simulink model "green_velocity"  (R2021a)
settings: Solver=VariableStepAuto  StartTime=0.0  StopTime=simTime  RelTol=1e-3
InitFcn:
  | gree_wave_velocity_init
values from neighbouring files (symbols this model uses):
  Kd = 0    [gree_wave_velocity_init.m]
  Ki = 51.1361    [gree_wave_velocity_init.m]
  Kp = 490.9572    [gree_wave_velocity_init.m]
  simTime = 1800    [gree_wave_velocity_init.m]
  v2x_traffic_signal = [light;time_fullwave(1:length(t)-1)]'    [gree_wave_velocity_init.m]
libraries: pid_lib x1
settings Model: Creator=srini  LastModifiedBy=srini

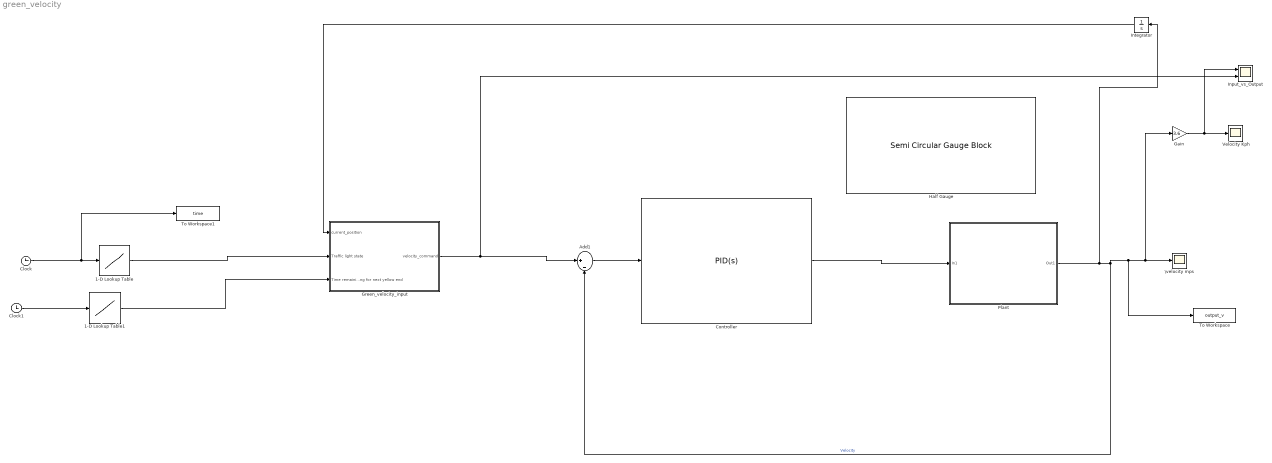
== system green_velocity ==
  1-D Lookup Table : Lookup_n-D  NumberOfTableDimensions=1  BreakpointsForDimension1=t(1:(simTime-1))  Table=v2x_traffic_signal(:,1)  InterpMethod=Nearest  InternalRulePriority=Speed  RndMeth=Simplest  InputSameDT=on
  1-D Lookup Table1 : Lookup_n-D  NumberOfTableDimensions=1  BreakpointsForDimension1=t(1:(simTime-1))  Table=v2x_traffic_signal(:,2)  InternalRulePriority=Speed  RndMeth=Simplest  InputSameDT=on
  Add1 : Sum  Inputs=|+-
  Clock : Clock
  Clock1 : Clock
  Controller : pid_lib/PID Controller  Controller=PID  Form=Parallel  TimeDomain=Continuous-time  UseExternalTs=off  SampleTime=-1  IntegratorMethod=Forward Euler  FilterMethod=Forward Euler  ControllerParametersSource=internal  P=Kp  I=Ki  D=Kd  UseFilter=on  N=100  TunerSelectOption=Transfer Function Based (PID Tuner App)  InitialConditionSource=internal  InitialConditionForIntegrator=0  InitialConditionForFilter=0  DifferentiatorICPrevScaledInput=0  ExternalReset=none  TrackingMode=off  Kt=1  LimitOutput=off  SatLimitsSource=internal  UpperSaturationLimit=inf  LowerSaturationLimit=-inf  LinearizeAsGain=on  AntiWindupMode=none  Kb=1  POutMin=[]  POutMax=[]  IOutMin=[]  IOutMax=[]  DOutMin=[]  DOutMax=[]  NOutMin=[]  NOutMax=[]  SumOutMin=[]  SumOutMax=[]  SaturationOutMin=[]  SaturationOutMax=[]  PParamMin=[]  PParamMax=[]  IParamMin=[]  IParamMax=[]  DParamMin=[]  DParamMax=[]  NParamMin=[]  NParamMax=[]  KbParamMin=[]  KbParamMax=[]  KtParamMin=[]  KtParamMax=[]  KbOutMin=[]  KbOutMax=[]  KtOutMin=[]  KtOutMax=[]  IntegratorOutMin=[]  IntegratorOutMax=[]  FilterOutMin=[]  FilterOutMax=[]  SumI1OutMin=[]  SumI1OutMax=[]  SumI2OutMin=[]  SumI2OutMax=[]  SumI3OutMin=[]  SumI3OutMax=[]  SumI4OutMin=[]  SumI4OutMax=[]  SumDOutMin=[]  SumDOutMax=[]  DifferentiatorOutMin=[]  DifferentiatorOutMax=[]  FilterDiffOutCoefMin=[]  FilterDiffOutCoefMax=[]  ReciprocalOutMin=[]  ReciprocalOutMax=[]  SumDenOutMin=[]  SumDenOutMax=[]  SumNumOutMin=[]  SumNumOutMax=[]  DivideOutMin=[]  DivideOutMax=[]  UdiffTsProdOutMin=[]  UdiffTsProdOutMax=[]  NTsProdOutMin=[]  NTsProdOutMax=[]  UintegralTsProdOutMin=[]  UintegralTsProdOutMax=[]  UngainTsProdOutMin=[]  UngainTsProdOutMax=[]  IntegratorContinuousStateAttributes=''  IntegratorStateMustResolveToSignalObject=off  IntegratorRTWStateStorageClass=Auto  FilterContinuousStateAttributes=''  FilterStateMustResolveToSignalObject=off  FilterRTWStateStorageClass=Auto  ParallelPVariant=InternalParameters  IdealPVariant=Disabled  IVariant=InternalParameters  DVariant=InternalParameters  IntegratorVariant=Continuous  SatVariant=Disabled  AWVariant=Passthrough  PCopyVariant=Disabled  TRVariant=Disabled  FdbkBlocksVariant=Forward  IdealPFdbkVariant=Disabled  SatFdbkVariant=Disabled  DerivativeFilterVariant=ContFilter  NVariant=InternalParameters  NCopyVariant=Disabled  FilterICVariant=InternalICsFilter  IntegratorICVariant=InternalICs  ExternalResetVariant=Disabled  TRSumVariant=Passthrough  SumFdbkVariant=Disabled  SumVariant=Sum_PID  TsampFilterVariant=InternalTs  TsampNgainVariant=Passthrough  TsampIntegralVariant=Passthrough  ExternalSaturationOutDataTypeStr=Inherit: Same as second input
  Gain : Gain  Gain=3.6
  Green_velocity_input : Subsystem
  Half Gauge : SemiCircularGaugeBlock
  Input_vs_Output : Scope  NumInputPorts=2
  Integrator : Integrator
  Plant : Subsystem
  To Workspace : ToWorkspace  VariableName=output_v  SampleTime=-1
  To Workspace1 : ToWorkspace  VariableName=time  SampleTime=-1
  Velocity Kph : Scope
  \velocity mps : Scope
  wires:
  Green_velocity_input/1(velocity_command) -> Add1/1, Input_vs_Output/2
  Add1/1 -> Controller/1
  Controller/1 -> Plant/1(In1)
  Gain/1 -> Input_vs_Output/1, Velocity Kph/1
  Plant/1(Out1) -> To Workspace/1, Gain/1, \velocity mps/1, Add1/2, Integrator/1  "Velocity"
  1-D Lookup Table/1 -> Green_velocity_input/2(Traffic light state)
  Clock/1 -> To Workspace1/1, 1-D Lookup Table/1
  Clock1/1 -> 1-D Lookup Table1/1
  1-D Lookup Table1/1 -> Green_velocity_input/3(Time remaining for next yellow end)
  Integrator/1 -> Green_velocity_input/1(current_position)

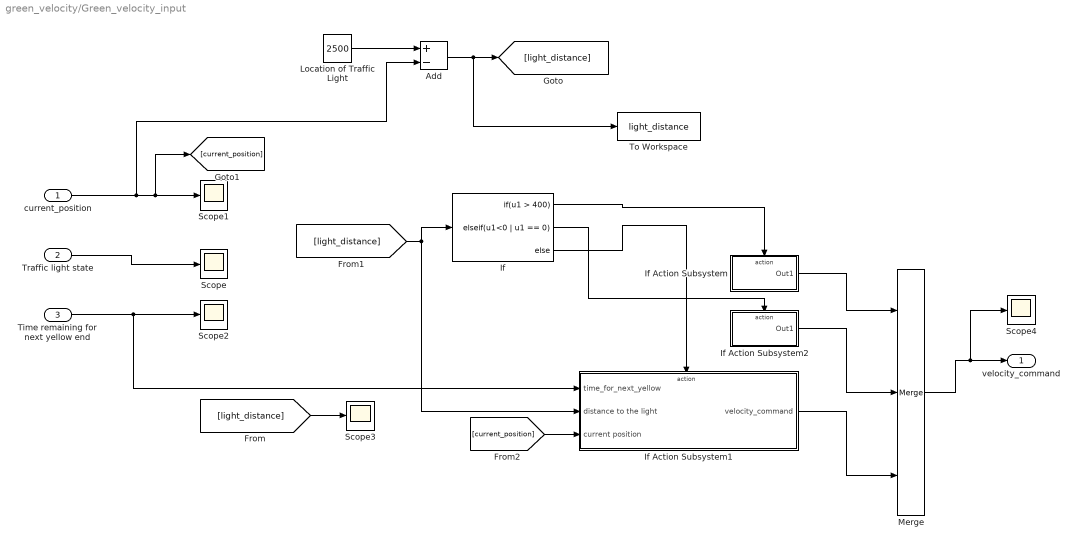
== system green_velocity/Green_velocity_input ==
  current_position : Inport
  Traffic light state : Inport  Port=2
  Time remaining for next yellow end : Inport  Port=3
  Add : Sum  Inputs=+-
  If : If  IfExpression=u1 > 400  ElseIfExpressions=u1<0 | u1 == 0
  If Action Subsystem : Subsystem  TreatAsAtomicUnit=on
  If Action Subsystem1 : Subsystem  TreatAsAtomicUnit=on
  If Action Subsystem2 : Subsystem  TreatAsAtomicUnit=on
  Location of Traffic Light : Constant  Value=2500
  Merge : Merge  Inputs=3
  Scope{,1..4} (5 alike) : Scope
  To Workspace : ToWorkspace  VariableName=light_distance  SampleTime=-1
  velocity_command : Outport
  wires:
  Traffic light state/1 -> Scope/1
  current_position/1 -> Add/2, [current_position], Scope1/1
  Location of Traffic Light/1 -> Add/1
  Add/1 -> To Workspace/1, [light_distance]
  Time remaining for next yellow end/1 -> If Action Subsystem1/1(time_for_next_yellow), Scope2/1
  [light_distance] -> Scope3/1
  [light_distance] -> If Action Subsystem1/2(distance to the light), If/1
  If/1 -> If Action Subsystem/Action
  If Action Subsystem/1(Out1) -> Merge/1
  Merge/1 -> Scope4/1, velocity_command/1
  If/3 -> If Action Subsystem1/Action
  If Action Subsystem1/1(velocity_command) -> Merge/3
  [current_position] -> If Action Subsystem1/3(current position)
  If/2 -> If Action Subsystem2/Action
  If Action Subsystem2/1(Out1) -> Merge/2

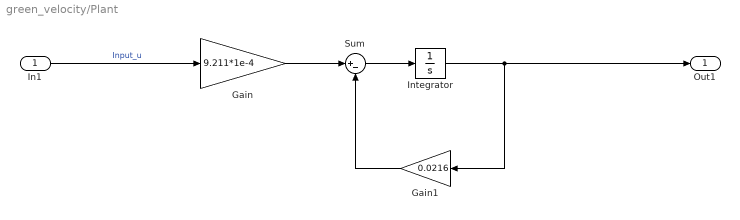
== system green_velocity/Plant ==
  In1 : Inport
  Gain : Gain  Gain=9.211*1e-4
  Gain1 : Gain  Gain=0.0216
  Integrator : Integrator  InitialCondition=15
  Sum : Sum  Inputs=|+-
  Out1 : Outport
  wires:
  Sum/1 -> Integrator/1
  Gain/1 -> Sum/1
  Gain1/1 -> Sum/2
  In1/1 -> Gain/1  "Input_u"
  Integrator/1 -> Out1/1, Gain1/1

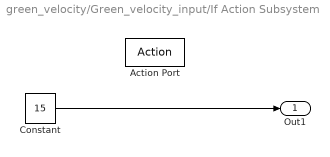
== system green_velocity/Green_velocity_input/If Action Subsystem ==
  Action Port : ActionPort  ActionPortLabel=if(u1 > 400)
  Constant : Constant  Value=15
  Out1 : Outport
  wires:
  Constant/1 -> Out1/1

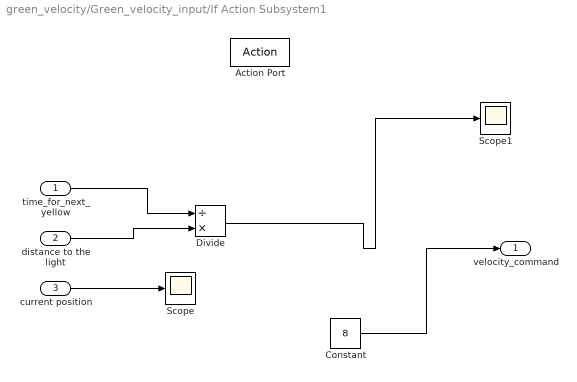
== system green_velocity/Green_velocity_input/If Action Subsystem1 ==
  time_for_next_yellow : Inport
  distance to the light : Inport  Port=2
  current position : Inport  Port=3
  Action Port : ActionPort  ActionPortLabel=else
  Constant : Constant  Value=8
  Divide : Product  Inputs=/*
  Scope : Scope
  Scope1 : Scope
  velocity_command : Outport
  wires:
  time_for_next_yellow/1 -> Divide/1
  distance to the light/1 -> Divide/2
  Divide/1 -> Scope1/1
  current position/1 -> Scope/1
  Constant/1 -> velocity_command/1

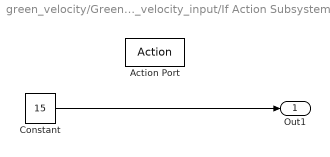
== system green_velocity/Green_velocity_input/If Action Subsystem2 ==
  Action Port : ActionPort  ActionPortLabel=elseif(u1<0 | u1 == 0)
  Constant : Constant  Value=15
  Out1 : Outport
  wires:
  Constant/1 -> Out1/1
